simulink model "PMSM_PI"  (R2024a)
settings: Solver=FixedStepAuto  StartTime=0.0  StopTime=10  FixedStep=TsModel  RelTol=1e-3
values from neighbouring files (symbols this model uses):
  ADRC_times = 4.0    [data_PMSM_PI.sldd]
  B = 0.0    [data_PMSM_PI.sldd]
  b0 = 2000.0    [data_PMSM_PI.sldd]
  CCR_Counter = 4199.0    [data_PMSM_PI.sldd]
  CUR_I = 105.0    [data_PMSM_PI.sldd]
  CUR_P = 0.255    [data_PMSM_PI.sldd]
  current_bandwidth = 1500.0    [data_PMSM_PI.sldd]
  currunt_omega_c = 350.0    [data_PMSM_PI.sldd]
  flux = 0.00419    [data_PMSM_PI.sldd]
  Idq_limit = 20.0    [data_PMSM_PI.sldd]
  J = 5.8E-5    [data_PMSM_PI.sldd]
  Ld = 0.00017    [data_PMSM_PI.sldd]
  Lq = 0.00017    [data_PMSM_PI.sldd]
  Ls = 0.00017    [data_PMSM_PI.sldd]
  omega_c = 330.0    [data_PMSM_PI.sldd]
  omega_c_LQR = 35.0    [data_PMSM_PI.sldd]
  PMSM_CCR_Counter = 4199.0    [data_PMSM_PI.sldd]
  Pn = 5.0    [data_PMSM_PI.sldd]
  Rs = 0.07    [data_PMSM_PI.sldd]
  speed_bandwidth = 200.0    [data_PMSM_PI.sldd]
  speed_bandwidth_LQR = 60.0    [data_PMSM_PI.sldd]
  SPEED_I = 18.457    [data_PMSM_PI.sldd]
  SPEED_P = 0.18457    [data_PMSM_PI.sldd]
  Ts = 0.0001    [data_PMSM_PI.sldd]
  TsModel = 2.5E-5    [data_PMSM_PI.sldd]
  two_b0 = 2649534.0    [data_PMSM_PI.sldd]
  two_omega_c = 85.0    [data_PMSM_PI.sldd]
undefined symbols (not defined in the file or in its folder): DiscIntNeverNeededParam, sigbuilder_block
libraries: slpidlib x4, simulink x1, mcbplantlib x1, autolibpmsmexterior x1
(part 2 of 2)

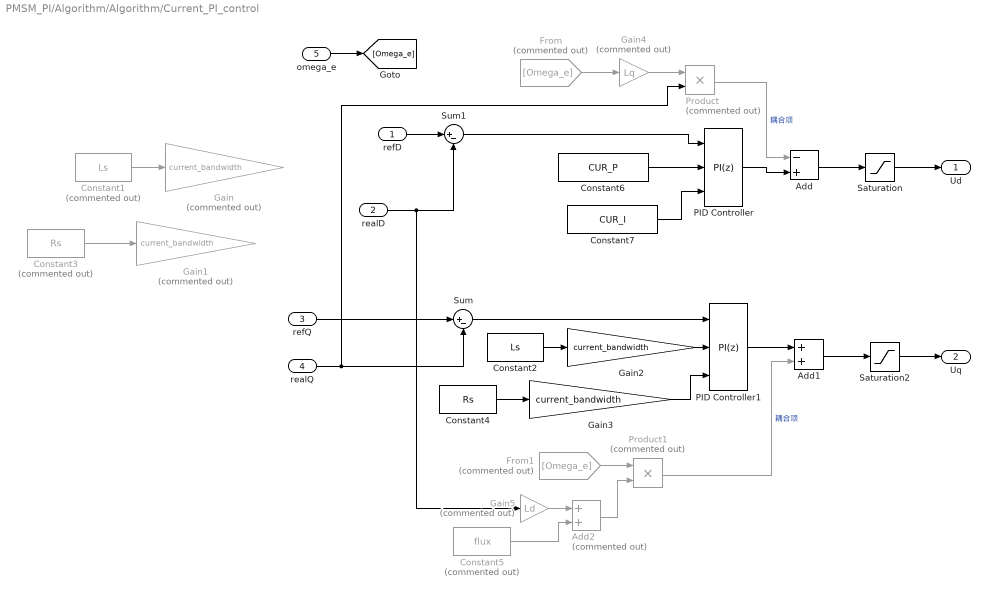
== system PMSM_PI/Algorithm/Algorithm/Current_PI_control ==
  refD : Inport  OutDataTypeStr=single
  realD : Inport  Port=2  OutDataTypeStr=single
  refQ : Inport  Port=3  OutDataTypeStr=single
  realQ : Inport  Port=4  OutDataTypeStr=single
  omega_e : Inport  Port=5  OutDataTypeStr=single
  Add : Sum  Inputs=-+  OutDataTypeStr=single
  Add1 : Sum  OutDataTypeStr=single
  Add2 : Sum  Commented=on  OutDataTypeStr=single
  Constant1 : Constant  Commented=on  Value=Ls  OutDataTypeStr=single  SampleTime=Ts
  Constant2 : Constant  Value=Ls  OutDataTypeStr=single  SampleTime=Ts
  Constant3 : Constant  Commented=on  Value=Rs  OutDataTypeStr=single  SampleTime=Ts
  Constant4 : Constant  Value=Rs  OutDataTypeStr=single  SampleTime=Ts
  Constant5 : Constant  Commented=on  Value=flux  OutDataTypeStr=single  SampleTime=Ts
  Constant6 : Constant  Value=CUR_P  OutDataTypeStr=single  SampleTime=Ts
  Constant7 : Constant  Value=CUR_I  OutDataTypeStr=single  SampleTime=Ts
  From : From  Commented=on  GotoTag=Omega_e
  From1 : From  Commented=on  GotoTag=Omega_e
  Gain : Gain  Commented=on  Gain=current_bandwidth  OutDataTypeStr=single
  Gain1 : Gain  Commented=on  Gain=current_bandwidth  OutDataTypeStr=single
  Gain2 : Gain  Gain=current_bandwidth  OutDataTypeStr=single
  Gain3 : Gain  Gain=current_bandwidth  OutDataTypeStr=single
  Gain4 : Gain  Commented=on  Gain=Lq  OutDataTypeStr=single
  Gain5 : Gain  Commented=on  Gain=Ld  OutDataTypeStr=single
  PID Controller : slpidlib/PID Controller  Controller=PI  Form=Parallel  TimeDomain=Discrete-time  UseExternalTs=off  SampleTime=Ts  IntegratorMethod=Forward Euler  FilterMethod=Forward Euler  ControllerParametersSource=external  P=1  I=1  UseKiTs=off  D=0  UseExternalDerivativeSource=off  N=100  UseFilter=on  TunerSelectOption=Transfer Function Based (PID Tuner App)  ZeroCross=off  InitialConditionSource=internal  InitialConditionForIntegrator=1  InitialConditionForFilter=0  DifferentiatorICPrevScaledInput=0  ExternalReset=none  TrackingMode=off  Kt=1  LimitOutput=off  SatLimitsSource=internal  UpperSaturationLimit=200  LowerSaturationLimit=-200  LinearizeAsGain=on  AntiWindupMode=none  Kb=1  LimitIntegrator=off  UpperIntegratorSaturationLimit=inf  LowerIntegratorSaturationLimit=-inf  POutMin=[]  POutMax=[]  IOutMin=[]  IOutMax=[]  DOutMin=[]  DOutMax=[]  NOutMin=[]  NOutMax=[]  SumOutMin=[]  SumOutMax=[]  SaturationOutMin=[]  SaturationOutMax=[]  PParamMin=[]  PParamMax=[]  IParamMin=[]  IParamMax=[]  DParamMin=[]  DParamMax=[]  NParamMin=[]  NParamMax=[]  KbParamMin=[]  KbParamMax=[]  KtParamMin=[]  KtParamMax=[]  KbOutMin=[]  KbOutMax=[]  KtOutMin=[]  KtOutMax=[]  IntegratorOutMin=[]  IntegratorOutMax=[]  FilterOutMin=[]  FilterOutMax=[]  SumI1OutMin=[]  SumI1OutMax=[]  SumI2OutMin=[]  SumI2OutMax=[]  SumI3OutMin=[]  SumI3OutMax=[]  SumI4OutMin=[]  SumI4OutMax=[]  SumDOutMin=[]  SumDOutMax=[]  DifferentiatorOutMin=[]  DifferentiatorOutMax=[]  FilterDiffOutCoefMin=[]  FilterDiffOutCoefMax=[]  ReciprocalOutMin=[]  ReciprocalOutMax=[]  SumDenOutMin=[]  SumDenOutMax=[]  SumNumOutMin=[]  SumNumOutMax=[]  DivideOutMin=[]  DivideOutMax=[]  UdiffTsProdOutMin=[]  UdiffTsProdOutMax=[]  NTsProdOutMin=[]  NTsProdOutMax=[]  UintegralTsProdOutMin=[]  UintegralTsProdOutMax=[]  UngainTsProdOutMin=[]  UngainTsProdOutMax=[]  ClampingZeroOutDataTypeStr=Inherit: Inherit via back propagation  ClampingZeroOutMin=[]  ClampingZeroOutMax=[]  FilterDenConstantOutDataTypeStr=Inherit: Inherit via back propagation  FilterDenConstantOutMin=[]  FilterDenConstantOutMax=[]  PCopyOutDataTypeStr=Inherit: Inherit via back propagation  PCopyOutMin=[]  PCopyOutMax=[]  NCopyOutDataTypeStr=Inherit: Inherit via back propagation  NCopyOutMin=[]  NCopyOutMax=[]  IntegratorContinuousStateAttributes=''  IntegratorStateMustResolveToSignalObject=off  IntegratorRTWStateStorageClass=Auto  FilterContinuousStateAttributes=''  FilterStateMustResolveToSignalObject=off  FilterRTWStateStorageClass=Auto  ParallelPVariant=ExternalParameters  IdealPVariant=Disabled  IVariant=ExternalParameters  DVariant=Disabled  IntegratorVariant=Discrete  SatVariant=Disabled  AWVariant=Passthrough  PCopyVariant=Disabled  TRVariant=Disabled  FdbkBlocksVariant=Forward  IdealPFdbkVariant=Disabled  SatFdbkVariant=Disabled  DerivativeFilterVariant=Disabled  NVariant=Disabled  NCopyVariant=Disabled_SignalSpec  FilterICVariant=Disabled  IntegratorICVariant=InternalICs  ExternalResetVariant=Disabled  TRSumVariant=Passthrough  SumFdbkVariant=Disabled  SumVariant=Sum_PI  TsampFilterVariant=InternalTs  TsampNgainVariant=Passthrough  TsampIntegralVariant=Disabled_SignalSpec  ExternalSaturationOutDataTypeStr=Inherit: Same as second input  DerivativeSourceVariant=Disabled
  PID Controller1 : slpidlib/PID Controller  Controller=PI  Form=Parallel  TimeDomain=Discrete-time  UseExternalTs=off  SampleTime=Ts  IntegratorMethod=Forward Euler  FilterMethod=Forward Euler  ControllerParametersSource=external  P=1  I=1  UseKiTs=off  D=0  UseExternalDerivativeSource=off  N=100  UseFilter=on  TunerSelectOption=Transfer Function Based (PID Tuner App)  ZeroCross=off  InitialConditionSource=internal  InitialConditionForIntegrator=1  InitialConditionForFilter=0  DifferentiatorICPrevScaledInput=0  ExternalReset=none  TrackingMode=off  Kt=1  LimitOutput=off  SatLimitsSource=internal  UpperSaturationLimit=200  LowerSaturationLimit=-200  LinearizeAsGain=on  AntiWindupMode=none  Kb=1  LimitIntegrator=off  UpperIntegratorSaturationLimit=inf  LowerIntegratorSaturationLimit=-inf  POutMin=[]  POutMax=[]  IOutMin=[]  IOutMax=[]  DOutMin=[]  DOutMax=[]  NOutMin=[]  NOutMax=[]  SumOutMin=[]  SumOutMax=[]  SaturationOutMin=[]  SaturationOutMax=[]  PParamMin=[]  PParamMax=[]  IParamMin=[]  IParamMax=[]  DParamMin=[]  DParamMax=[]  NParamMin=[]  NParamMax=[]  KbParamMin=[]  KbParamMax=[]  KtParamMin=[]  KtParamMax=[]  KbOutMin=[]  KbOutMax=[]  KtOutMin=[]  KtOutMax=[]  IntegratorOutMin=[]  IntegratorOutMax=[]  FilterOutMin=[]  FilterOutMax=[]  SumI1OutMin=[]  SumI1OutMax=[]  SumI2OutMin=[]  SumI2OutMax=[]  SumI3OutMin=[]  SumI3OutMax=[]  SumI4OutMin=[]  SumI4OutMax=[]  SumDOutMin=[]  SumDOutMax=[]  DifferentiatorOutMin=[]  DifferentiatorOutMax=[]  FilterDiffOutCoefMin=[]  FilterDiffOutCoefMax=[]  ReciprocalOutMin=[]  ReciprocalOutMax=[]  SumDenOutMin=[]  SumDenOutMax=[]  SumNumOutMin=[]  SumNumOutMax=[]  DivideOutMin=[]  DivideOutMax=[]  UdiffTsProdOutMin=[]  UdiffTsProdOutMax=[]  NTsProdOutMin=[]  NTsProdOutMax=[]  UintegralTsProdOutMin=[]  UintegralTsProdOutMax=[]  UngainTsProdOutMin=[]  UngainTsProdOutMax=[]  ClampingZeroOutDataTypeStr=Inherit: Inherit via back propagation  ClampingZeroOutMin=[]  ClampingZeroOutMax=[]  FilterDenConstantOutDataTypeStr=Inherit: Inherit via back propagation  FilterDenConstantOutMin=[]  FilterDenConstantOutMax=[]  PCopyOutDataTypeStr=Inherit: Inherit via back propagation  PCopyOutMin=[]  PCopyOutMax=[]  NCopyOutDataTypeStr=Inherit: Inherit via back propagation  NCopyOutMin=[]  NCopyOutMax=[]  IntegratorContinuousStateAttributes=''  IntegratorStateMustResolveToSignalObject=off  IntegratorRTWStateStorageClass=Auto  FilterContinuousStateAttributes=''  FilterStateMustResolveToSignalObject=off  FilterRTWStateStorageClass=Auto  ParallelPVariant=ExternalParameters  IdealPVariant=Disabled  IVariant=ExternalParameters  DVariant=Disabled  IntegratorVariant=Discrete  SatVariant=Disabled  AWVariant=Passthrough  PCopyVariant=Disabled  TRVariant=Disabled  FdbkBlocksVariant=Forward  IdealPFdbkVariant=Disabled  SatFdbkVariant=Disabled  DerivativeFilterVariant=Disabled  NVariant=Disabled  NCopyVariant=Disabled_SignalSpec  FilterICVariant=Disabled  IntegratorICVariant=InternalICs  ExternalResetVariant=Disabled  TRSumVariant=Passthrough  SumFdbkVariant=Disabled  SumVariant=Sum_PI  TsampFilterVariant=InternalTs  TsampNgainVariant=Passthrough  TsampIntegralVariant=Disabled_SignalSpec  ExternalSaturationOutDataTypeStr=Inherit: Same as second input  DerivativeSourceVariant=Disabled
  Product : Product  Commented=on  OutDataTypeStr=single
  Product1 : Product  Commented=on  OutDataTypeStr=single
  Saturation : Saturate  UpperLimit=Idq_limit  LowerLimit=-Idq_limit  OutDataTypeStr=single
  Saturation2 : Saturate  UpperLimit=Idq_limit  LowerLimit=-Idq_limit  OutDataTypeStr=single
  Sum : Sum  Inputs=|+-  OutDataTypeStr=single
  Sum1 : Sum  Inputs=|+-  OutDataTypeStr=single
  Ud : Outport  OutDataTypeStr=single
  Uq : Outport  Port=2  OutDataTypeStr=single
  wires:
  realD/1 -> Gain5/1, Sum1/2
  realQ/1 -> Product/2, Sum/2
  Add1/1 -> Saturation2/1
  Saturation/1 -> Ud/1
  Sum/1 -> PID Controller1/1
  Sum1/1 -> PID Controller/1
  refD/1 -> Sum1/1
  refQ/1 -> Sum/1
  Constant2/1 -> Gain2/1
  Gain3/1 -> PID Controller1/3
  Gain2/1 -> PID Controller1/2
  Constant1/1 -> Gain/1
  Constant4/1 -> Gain3/1
  Constant3/1 -> Gain1/1
  PID Controller/1 -> Add/2
  Add/1 -> Saturation/1
  omega_e/1 -> [Omega_e]
  From/1 -> Gain4/1
  Gain4/1 -> Product/1
  Product/1 -> Add/1  "耦合项"
  PID Controller1/1 -> Add1/1
  From1/1 -> Product1/1
  Gain5/1 -> Add2/1
  Constant5/1 -> Add2/2
  Add2/1 -> Product1/2
  Product1/1 -> Add1/2  "耦合项"
  Saturation2/1 -> Uq/1
  Constant6/1 -> PID Controller/2
  Constant7/1 -> PID Controller/3

== system PMSM_PI/Algorithm/Algorithm/Currunt_LADRC_Control ==
  Id_ref : Inport
  Id_real : Inport  Port=2
  Iq_ref : Inport  Port=3
  Iq_real : Inport  Port=4
  omega_e : Inport  Port=5
  Add3 : Sum  Inputs=-+  OutDataTypeStr=single
  Add4 : Sum  OutDataTypeStr=single
  Add5 : Sum  Commented=on  OutDataTypeStr=single
  Constant6 : Constant  Commented=on  Value=flux  OutDataTypeStr=single  SampleTime=Ts
  From12 : From  Commented=on  GotoTag=Omega_e
  From13 : From  Commented=on  GotoTag=Omega_e
  Gain6 : Gain  Commented=on  Gain=Lq  OutDataTypeStr=single
  Gain7 : Gain  Commented=on  Gain=Ld  OutDataTypeStr=single
  Id_Currunt_LADRC_Control : Subsystem
  Iq_Currunt_LADRC_Control : Subsystem
  Product2 : Product  Commented=on  OutDataTypeStr=single
  Product3 : Product  Commented=on  OutDataTypeStr=single
  Saturation1 : Saturate  UpperLimit=Idq_limit  LowerLimit=-Idq_limit  OutDataTypeStr=single
  Saturation3 : Saturate  UpperLimit=Idq_limit  LowerLimit=-Idq_limit  OutDataTypeStr=single
  ud_Ref : Outport
  uq_Ref : Outport  Port=2
  wires:
  Id_Currunt_LADRC_Control/1(ud_Ref) -> Add3/2
  Id_real/1 -> Gain7/1, Id_Currunt_LADRC_Control/2(Id_real)
  Product2/1 -> Add3/1  "耦合项"
  Constant6/1 -> Add5/2
  Product3/1 -> Add4/2  "耦合项"
  Id_ref/1 -> Id_Currunt_LADRC_Control/1(Id_ref)
  Add5/1 -> Product3/2
  Add3/1 -> Saturation1/1
  Iq_Currunt_LADRC_Control/1(uq_Ref) -> Add4/1
  Gain7/1 -> Add5/1
  Add4/1 -> Saturation3/1
  From12/1 -> Product3/1
  From13/1 -> Gain6/1
  Iq_ref/1 -> Iq_Currunt_LADRC_Control/1(Iq_ref)
  Iq_real/1 -> Product2/2, Iq_Currunt_LADRC_Control/2(Iq_real)
  Gain6/1 -> Product2/1
  Saturation1/1 -> ud_Ref/1
  Saturation3/1 -> uq_Ref/1
  omega_e/1 -> [Omega_e]

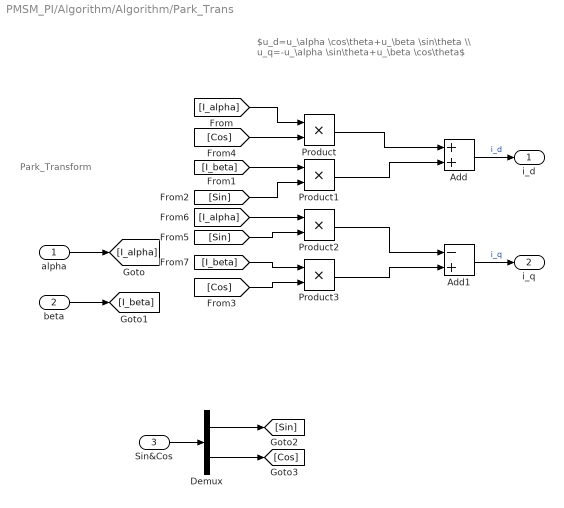
== system PMSM_PI/Algorithm/Algorithm/Park_Trans ==
  note: $u_d=u_\alpha \cos\theta+u_\beta \sin\theta \\ u_q=-u_\alpha \sin\theta+u_\beta \cos\theta$
  note: Park_Transform
  alpha : Inport  OutDataTypeStr=single
  beta : Inport  Port=2  OutDataTypeStr=single
  Sin&Cos : Inport  Port=3  OutDataTypeStr=single
  Add : Sum  OutDataTypeStr=single
  Add1 : Sum  Inputs=-+  OutDataTypeStr=single
  Demux : Demux  Outputs=2
  Product{,1..3} (4 alike) : Product  OutDataTypeStr=single
  i_d : Outport  OutDataTypeStr=single
  i_q : Outport  Port=2  OutDataTypeStr=single
  wires:
  Add1/1 -> i_q/1  "i_q"
  [Cos] -> Product/2
  Product/1 -> Add/1
  Product1/1 -> Add/2
  beta/1 -> [I_beta]
  Add/1 -> i_d/1  "i_d"
  [I_alpha] -> Product/1
  Product3/1 -> Add1/2
  [I_beta] -> Product3/1
  [I_beta] -> Product1/1
  [Sin] -> Product2/2
  Product2/1 -> Add1/1
  [Sin] -> Product1/2
  [I_alpha] -> Product2/1
  alpha/1 -> [I_alpha]
  [Cos] -> Product3/2
  Demux/1 -> [Sin]
  Demux/2 -> [Cos]
  Sin&Cos/1 -> Demux/1

== system PMSM_PI/Algorithm/Algorithm/SVPWM_By_Average_Zero_Injection ==
  d : Inport  OutDataTypeStr=single
  q : Inport  Port=2  OutDataTypeStr=single
  Sin&Cos : Inport  Port=3  OutDataTypeStr=single
  Udc : Inport  Port=4  OutDataTypeStr=single
  Anti_Park_Trans : Subsystem
  Gain : Gain  Gain=CCR_Counter  OutDataTypeStr=single
  Gain1 : Gain  Gain=CCR_Counter  OutDataTypeStr=single
  Gain2 : Gain  Gain=CCR_Counter  OutDataTypeStr=single
  SVPWM : Subsystem
  Scope : Scope  NumInputPorts=3
  Ta : Outport  OutDataTypeStr=single
  Tb : Outport  Port=2  OutDataTypeStr=single
  Tc : Outport  Port=3  OutDataTypeStr=single
  U_alpha : Outport  Port=4  OutDataTypeStr=single
  U_beta : Outport  Port=5  OutDataTypeStr=single
  wires:
  Anti_Park_Trans/1(alpha) -> U_alpha/1, SVPWM/1(alpha)
  q/1 -> Anti_Park_Trans/2(q)
  SVPWM/1(Ta) -> Scope/1, Gain/1
  Anti_Park_Trans/2(beta) -> U_beta/1, SVPWM/2(beta)
  d/1 -> Anti_Park_Trans/1(d)
  Sin&Cos/1 -> Anti_Park_Trans/3(Sin&Cos)
  SVPWM/2(Tb) -> Scope/2, Gain1/1
  SVPWM/3(Tc) -> Gain2/1, Scope/3
  Udc/1 -> SVPWM/3(Udc)
  Gain/1 -> Ta/1
  Gain1/1 -> Tb/1
  Gain2/1 -> Tc/1

== system PMSM_PI/Algorithm/Algorithm/Speed PI control2 ==
  Ref_RPM : Inport  OutDataTypeStr=single
  Real_RPM : Inport  Port=2  OutDataTypeStr=single
  Add : Sum  Inputs=+-  OutDataTypeStr=single
  Constant1 : Constant  Commented=on  Value=speed_bandwidth  OutDataTypeStr=single  SampleTime=Ts
  Constant2 : Constant  Value=speed_bandwidth  OutDataTypeStr=single  SampleTime=Ts
  Constant3 : Constant  Value=B  OutDataTypeStr=single  SampleTime=Ts
  Constant4 : Constant  Value=1.5*Pn*flux  OutDataTypeStr=single  SampleTime=Ts
  Constant5 : Constant  Value=SPEED_P  OutDataTypeStr=single  SampleTime=Ts
  Constant6 : Constant  Value=SPEED_I  OutDataTypeStr=single  SampleTime=Ts
  Divide : Product  Inputs=*/  OutDataTypeStr=single
  Gain : Gain  Commented=on  Gain=J/(1.5*Pn*flux)  OutDataTypeStr=single
  Gain1 : Gain  Commented=on  Gain=J/(1.5*Pn*flux)  OutDataTypeStr=single
  Gain2 : Gain  Gain=J  OutDataTypeStr=single
  PID Controller : slpidlib/PID Controller  Controller=PI  Form=Parallel  TimeDomain=Discrete-time  UseExternalTs=off  SampleTime=Ts  IntegratorMethod=Forward Euler  FilterMethod=Forward Euler  ControllerParametersSource=external  P=1  I=1  UseKiTs=off  D=0  UseExternalDerivativeSource=off  N=100  UseFilter=on  TunerSelectOption=Transfer Function Based (PID Tuner App)  ZeroCross=off  InitialConditionSource=internal  InitialConditionForIntegrator=1  InitialConditionForFilter=0  DifferentiatorICPrevScaledInput=0  ExternalReset=none  TrackingMode=off  Kt=1  LimitOutput=off  SatLimitsSource=internal  UpperSaturationLimit=200  LowerSaturationLimit=-200  LinearizeAsGain=on  AntiWindupMode=none  Kb=1  LimitIntegrator=off  UpperIntegratorSaturationLimit=inf  LowerIntegratorSaturationLimit=-inf  POutMin=[]  POutMax=[]  IOutMin=[]  IOutMax=[]  DOutMin=[]  DOutMax=[]  NOutMin=[]  NOutMax=[]  SumOutMin=[]  SumOutMax=[]  SaturationOutMin=[]  SaturationOutMax=[]  PParamMin=[]  PParamMax=[]  IParamMin=[]  IParamMax=[]  DParamMin=[]  DParamMax=[]  NParamMin=[]  NParamMax=[]  KbParamMin=[]  KbParamMax=[]  KtParamMin=[]  KtParamMax=[]  KbOutMin=[]  KbOutMax=[]  KtOutMin=[]  KtOutMax=[]  IntegratorOutMin=[]  IntegratorOutMax=[]  FilterOutMin=[]  FilterOutMax=[]  SumI1OutMin=[]  SumI1OutMax=[]  SumI2OutMin=[]  SumI2OutMax=[]  SumI3OutMin=[]  SumI3OutMax=[]  SumI4OutMin=[]  SumI4OutMax=[]  SumDOutMin=[]  SumDOutMax=[]  DifferentiatorOutMin=[]  DifferentiatorOutMax=[]  FilterDiffOutCoefMin=[]  FilterDiffOutCoefMax=[]  ReciprocalOutMin=[]  ReciprocalOutMax=[]  SumDenOutMin=[]  SumDenOutMax=[]  SumNumOutMin=[]  SumNumOutMax=[]  DivideOutMin=[]  DivideOutMax=[]  UdiffTsProdOutMin=[]  UdiffTsProdOutMax=[]  NTsProdOutMin=[]  NTsProdOutMax=[]  UintegralTsProdOutMin=[]  UintegralTsProdOutMax=[]  UngainTsProdOutMin=[]  UngainTsProdOutMax=[]  ClampingZeroOutDataTypeStr=Inherit: Inherit via back propagation  ClampingZeroOutMin=[]  ClampingZeroOutMax=[]  FilterDenConstantOutDataTypeStr=Inherit: Inherit via back propagation  FilterDenConstantOutMin=[]  FilterDenConstantOutMax=[]  PCopyOutDataTypeStr=Inherit: Inherit via back propagation  PCopyOutMin=[]  PCopyOutMax=[]  NCopyOutDataTypeStr=Inherit: Inherit via back propagation  NCopyOutMin=[]  NCopyOutMax=[]  IntegratorContinuousStateAttributes=''  IntegratorStateMustResolveToSignalObject=off  IntegratorRTWStateStorageClass=Auto  FilterContinuousStateAttributes=''  FilterStateMustResolveToSignalObject=off  FilterRTWStateStorageClass=Auto  ParallelPVariant=ExternalParameters  IdealPVariant=Disabled  IVariant=ExternalParameters  DVariant=Disabled  IntegratorVariant=Discrete  SatVariant=Disabled  AWVariant=Passthrough  PCopyVariant=Disabled  TRVariant=Disabled  FdbkBlocksVariant=Forward  IdealPFdbkVariant=Disabled  SatFdbkVariant=Disabled  DerivativeFilterVariant=Disabled  NVariant=Disabled  NCopyVariant=Disabled_SignalSpec  FilterICVariant=Disabled  IntegratorICVariant=InternalICs  ExternalResetVariant=Disabled  TRSumVariant=Passthrough  SumFdbkVariant=Disabled  SumVariant=Sum_PI  TsampFilterVariant=InternalTs  TsampNgainVariant=Passthrough  TsampIntegralVariant=Disabled_SignalSpec  ExternalSaturationOutDataTypeStr=Inherit: Same as second input  DerivativeSourceVariant=Disabled
  Product : Product  Commented=on  OutDataTypeStr=single
  Product1 : Product  OutDataTypeStr=single
  Saturation2 : Saturate  UpperLimit=Idq_limit  LowerLimit=-Idq_limit  OutDataTypeStr=single
  Sum1 : Sum  Inputs=|+-  OutDataTypeStr=single
  Sum2 : Sum  Inputs=|+-  OutDataTypeStr=single
  Iq_out : Outport  OutDataTypeStr=single
  wires:
  Constant1/1 -> Gain/1
  Ref_RPM/1 -> Sum1/1
  Sum1/1 -> PID Controller/1
  Real_RPM/1 -> Product1/2, Sum1/2
  PID Controller/1 -> Sum2/1
  Constant2/1 -> Product/1, Product/2, Gain2/1
  Product/1 -> Gain1/1
  Gain2/1 -> Add/1
  Constant3/1 -> Add/2
  Add/1 -> Divide/1
  Constant4/1 -> Divide/2
  Divide/1 -> Product1/1
  Product1/1 -> Sum2/2
  Saturation2/1 -> Iq_out/1
  Sum2/1 -> Saturation2/1
  Constant5/1 -> PID Controller/2
  Constant6/1 -> PID Controller/3

== system PMSM_PI/Algorithm/Algorithm/Speed SMC control1 ==
  note: 机械转速（rad/s）
  note: 转速值（单位RPM）
  Ref_RPM : Inport  OutDataTypeStr=single
  Real_RPM : Inport  Port=2  OutDataTypeStr=single
  1/D : Gain  Gain=1/(1.5*Pn*flux/2/J)  SaturateOnIntegerOverflow=on  SampleTime=Ts  OutDataTypeStr=Inherit: Same as input  ParamDataTypeStr=Inherit: Same as input
  Discrete Derivative : simulink/Discrete/Discrete Derivative  gainval=1.0  ICPrevScaledInput=0.0  OutMin=[]  OutMax=[]  OutDataType=fixdt(1, 16)  OutScaling=2^-10  DoSatur=off
  Discrete-Time Integrator : DiscreteIntegrator  InitialCondition=0.001  SampleTime=Ts  ICPrevOutput=DiscIntNeverNeededParam  ICPrevScaledInput=DiscIntNeverNeededParam
  Kp1 : Gain  Gain=300  SaturateOnIntegerOverflow=on  SampleTime=Ts  OutDataTypeStr=Inherit: Same as input  ParamDataTypeStr=Inherit: Same as input
  Kp2 : Gain  Gain=200  SaturateOnIntegerOverflow=on  SampleTime=Ts  OutDataTypeStr=Inherit: Same as input  ParamDataTypeStr=Inherit: Same as input
  Kp3 : Gain  Gain=60  SaturateOnIntegerOverflow=on  SampleTime=Ts  OutDataTypeStr=Inherit: Same as input  ParamDataTypeStr=Inherit: Same as input
  Kp4 : Gain  Gain=60  SaturateOnIntegerOverflow=on  SampleTime=Ts  OutDataTypeStr=Inherit: Same as input  ParamDataTypeStr=Inherit: Same as input
  Nr->wm : Gain  Gain=pi/30  SaturateOnIntegerOverflow=on  SampleTime=Ts  OutDataTypeStr=Inherit: Same as input  ParamDataTypeStr=Inherit: Same as input
  Saturation2 : Saturate  UpperLimit=Idq_limit  LowerLimit=-Idq_limit  OutDataTypeStr=single
  Sign : Signum
  Sum1 : Sum  Inputs=|+-  OutDataTypeStr=single
  Sum3 : Sum  InputSameDT=on  SaturateOnIntegerOverflow=on  SampleTime=Ts  OutDataTypeStr=Inherit: Same as first input
  Sum4 : Sum  Inputs=++-  InputSameDT=on  SaturateOnIntegerOverflow=on  SampleTime=Ts  OutDataTypeStr=Inherit: Same as first input
  Iq_out : Outport  OutDataTypeStr=single
  wires:
  Ref_RPM/1 -> Sum1/1
  Real_RPM/1 -> Sum1/2
  Saturation2/1 -> Iq_out/1
  Discrete-Time Integrator/1 -> 1/D/1
  Sign/1 -> Kp2/1
  Kp1/1 -> Sum4/1
  Kp3/1 -> Sum4/3
  Kp4/1 -> Sum3/1
  Sum4/1 -> Discrete-Time Integrator/1
  Sum1/1 -> Nr->wm/1
  Sum3/1 -> Sign/1, Kp1/1
  Discrete Derivative/1 -> Kp3/1, Sum3/2  "x2"
  Kp2/1 -> Sum4/2
  Nr->wm/1 -> Discrete Derivative/1, Kp4/1  "x1"
  1/D/1 -> Saturation2/1

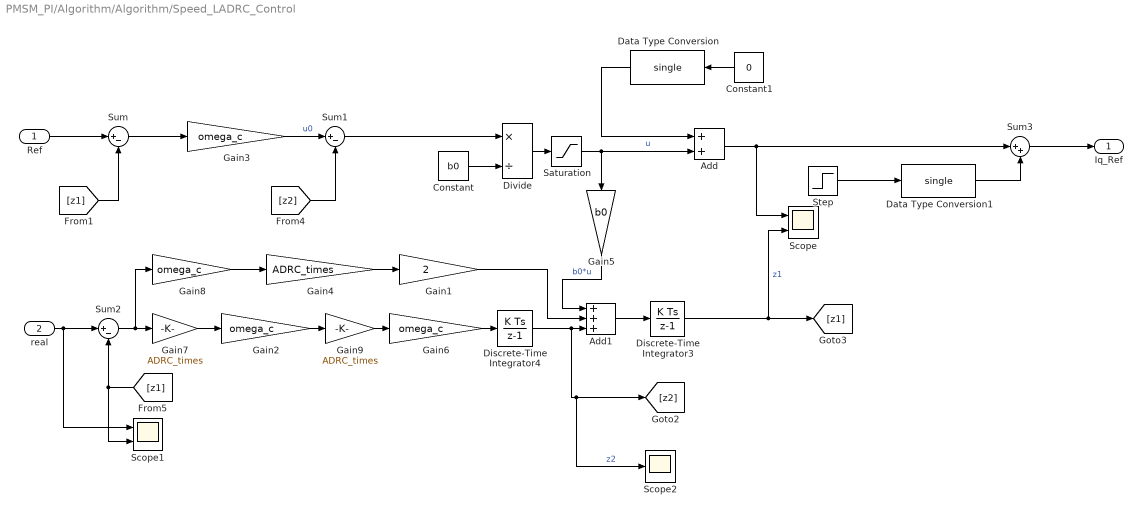
== system PMSM_PI/Algorithm/Algorithm/Speed_LADRC_Control ==
  Ref : Inport  OutDataTypeStr=single
  real : Inport  Port=2  OutDataTypeStr=single
  Add : Sum  OutDataTypeStr=single
  Add1 : Sum  Inputs=+++  OutDataTypeStr=single
  Constant : Constant  Value=b0  OutDataTypeStr=single
  Constant1 : Constant  Value=0  SampleTime=-1
  Data Type Conversion : DataTypeConversion  OutDataTypeStr=single  SaturateOnIntegerOverflow=off  RndMeth=Floor
  Data Type Conversion1 : DataTypeConversion  OutDataTypeStr=single  SaturateOnIntegerOverflow=off  RndMeth=Floor
  Discrete-Time Integrator3 : DiscreteIntegrator  SampleTime=-1  OutDataTypeStr=single  ICPrevOutput=DiscIntNeverNeededParam  ICPrevScaledInput=DiscIntNeverNeededParam
  Discrete-Time Integrator4 : DiscreteIntegrator  SampleTime=-1  OutDataTypeStr=single  ICPrevOutput=DiscIntNeverNeededParam  ICPrevScaledInput=DiscIntNeverNeededParam
  Divide : Product  Inputs=*/  OutDataTypeStr=single
  Gain1 : Gain  Gain=2  OutDataTypeStr=single
  Gain{2..3,6,8} (4 alike) : Gain  Gain=omega_c  OutDataTypeStr=single
  Gain4 : Gain  Gain=ADRC_times  OutDataTypeStr=single
  Gain5 : Gain  Gain=b0  OutDataTypeStr=single
  Gain7 : Gain  Gain=ADRC_times  OutDataTypeStr=single
  Gain9 : Gain  Gain=ADRC_times  OutDataTypeStr=single
  Saturation : Saturate  UpperLimit=Idq_limit  LowerLimit=-Idq_limit  OutDataTypeStr=single
  Scope : Scope  NumInputPorts=2
  Scope1 : Scope  NumInputPorts=2
  Scope2 : Scope
  Step : Step  Time=8  SampleTime=0
  Sum : Sum  Inputs=|+-  OutDataTypeStr=single
  Sum1 : Sum  Inputs=|+-  OutDataTypeStr=single
  Sum2 : Sum  Inputs=|+-  OutDataTypeStr=single
  Sum3 : Sum  Inputs=|++
  Iq_Ref : Outport  OutDataTypeStr=single
  wires:
  Ref/1 -> Sum/1
  Discrete-Time Integrator4/1 -> Add1/3, Scope2/1, [z2]  "z2"
  Gain5/1 -> Add1/1  "b0*u"
  Gain2/1 -> Gain9/1
  Gain1/1 -> Add1/2
  Discrete-Time Integrator3/1 -> Scope/2, [z1]  "z1"
  Add1/1 -> Discrete-Time Integrator3/1
  Sum2/1 -> Gain7/1, Gain8/1
  real/1 -> Scope1/1, Sum2/1
  [z1] -> Scope1/2, Sum2/2
  [z1] -> Sum/2
  Sum/1 -> Gain3/1
  [z2] -> Sum1/2
  Constant/1 -> Divide/2
  Divide/1 -> Saturation/1
  Gain3/1 -> Sum1/1  "u0"
  Sum1/1 -> Divide/1
  Add/1 -> Scope/1, Sum3/1
  Data Type Conversion/1 -> Add/1
  Saturation/1 -> Add/2, Gain5/1  "u"
  Gain4/1 -> Gain1/1
  Gain6/1 -> Discrete-Time Integrator4/1
  Gain7/1 -> Gain2/1
  Gain8/1 -> Gain4/1
  Gain9/1 -> Gain6/1
  Constant1/1 -> Data Type Conversion/1
  Sum3/1 -> Iq_Ref/1
  Step/1 -> Data Type Conversion1/1
  Data Type Conversion1/1 -> Sum3/2

== system PMSM_PI/Algorithm/Algorithm/Subsystem1 ==
  rpm_ref : Inport
  rpm_real : Inport  Port=2
  Id_ref : Inport  Port=3
  Id_real : Inport  Port=4
  Id_Currunt_LADRC_Control : Subsystem
  Subsystem : Subsystem
  uq_ref : Outport
  ud_Ref : Outport  Port=2
  wires:
  Id_Currunt_LADRC_Control/1(ud_Ref) -> ud_Ref/1
  Id_real/1 -> Id_Currunt_LADRC_Control/2(Id_real)
  Id_ref/1 -> Id_Currunt_LADRC_Control/1(Id_ref)
  rpm_ref/1 -> Subsystem/1(rpm_ref)
  rpm_real/1 -> Subsystem/2(rpm_real)
  Subsystem/1(uq_ref) -> uq_ref/1

== system PMSM_PI/Algorithm/Algorithm/Theta_to_SinCos ==
  Theta_in : Inport  OutDataTypeStr=single
  Mux : Mux  Inputs=2
  Sin : Trigonometry
  Sin1 : Trigonometry  Operator=cos
  Sin&Cos : Outport  OutDataTypeStr=single
  wires:
  Theta_in/1 -> Sin1/1, Sin/1
  Sin/1 -> Mux/1
  Sin1/1 -> Mux/2
  Mux/1 -> Sin&Cos/1

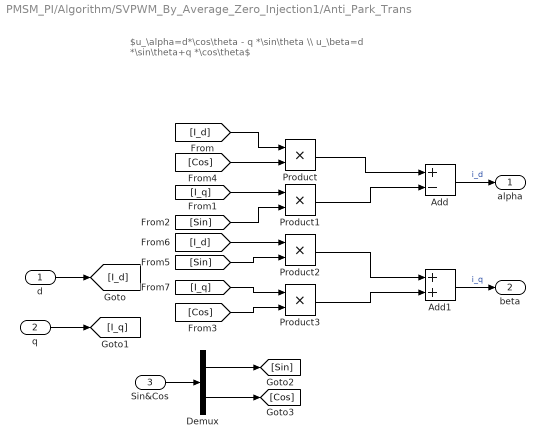
== system PMSM_PI/Algorithm/SVPWM_By_Average_Zero_Injection1/Anti_Park_Trans ==
  note: $u_\alpha=d*\cos\theta - q *\sin\theta \\ u_\beta=d *\sin\theta+q *\cos\theta$
  d : Inport  OutDataTypeStr=single
  q : Inport  Port=2  OutDataTypeStr=single
  Sin&Cos : Inport  Port=3  OutDataTypeStr=single
  Add : Sum  Inputs=+-  OutDataTypeStr=single
  Add1 : Sum  OutDataTypeStr=single
  Demux : Demux  Outputs=2
  Product{,1..3} (4 alike) : Product  OutDataTypeStr=single
  alpha : Outport  OutDataTypeStr=single
  beta : Outport  Port=2  OutDataTypeStr=single
  wires:
  Add1/1 -> beta/1  "i_q"
  Sin&Cos/1 -> Demux/1
  [Cos] -> Product/2
  Product/1 -> Add/1
  Product1/1 -> Add/2
  q/1 -> [I_q]
  Add/1 -> alpha/1  "i_d"
  [I_d] -> Product/1
  Product3/1 -> Add1/2
  [I_q] -> Product3/1
  [I_q] -> Product1/1
  [Sin] -> Product2/2
  Product2/1 -> Add1/1
  [Sin] -> Product1/2
  [I_d] -> Product2/1
  d/1 -> [I_d]
  [Cos] -> Product3/2
  Demux/1 -> [Sin]
  Demux/2 -> [Cos]

== system PMSM_PI/Algorithm/SVPWM_By_Average_Zero_Injection1/SVPWM ==
  alpha : Inport  OutDataTypeStr=single
  beta : Inport  Port=2  OutDataTypeStr=single
  Udc : Inport  Port=3  OutDataTypeStr=single
  Add{,1..4} (5 alike) : Sum  OutDataTypeStr=single
  Anti_Clark_Trans : Subsystem
  Constant : Constant  Value=0.5  OutDataTypeStr=single  SampleTime=Ts
  Demux : Demux  Outputs=3
  Divide : Product  Inputs=*/  OutDataTypeStr=single
  Gain : Gain  Gain=-0.5  OutDataTypeStr=single
  Gain1 : Gain  Gain=-1
  Max : MinMax  Function=max  Inputs=3  OutDataTypeStr=single
  Max1 : MinMax  Inputs=3  OutDataTypeStr=single
  Mux : Mux  Inputs=3
  Scope : Scope  NumInputPorts=3
  Ta : Outport  OutDataTypeStr=single
  Tb : Outport  Port=2  OutDataTypeStr=single
  Tc : Outport  Port=3  OutDataTypeStr=single
  wires:
  Anti_Clark_Trans/1(A) -> Max1/1, Max/1, Add/1
  Gain/1 -> Add/2, Add1/2, Add2/2
  Anti_Clark_Trans/2(B) -> Max1/2, Max/2, Add1/1
  Anti_Clark_Trans/3(C) -> Max1/3, Max/3, Add2/1
  Add3/1 -> Gain/1
  Max/1 -> Add3/1
  alpha/1 -> Anti_Clark_Trans/1(alpha)
  beta/1 -> Anti_Clark_Trans/2(beta)
  Add/1 -> Mux/1
  Add1/1 -> Mux/2
  Add2/1 -> Mux/3
  Mux/1 -> Gain1/1
  Demux/1 -> Ta/1
  Demux/2 -> Tb/1
  Demux/3 -> Tc/1
  Divide/1 -> Scope/2, Add4/1
  Constant/1 -> Add4/2
  Max1/1 -> Add3/2
  Udc/1 -> Divide/2
  Add4/1 -> Demux/1, Scope/3
  Gain1/1 -> Scope/1, Divide/1

== system PMSM_PI/Algorithm/Algorithm/Currunt_LADRC_Control/Id_Currunt_LADRC_Control ==
  Id_ref : Inport
  Id_real : Inport  Port=2
  Add1 : Sum  Inputs=+++
  Constant : Constant  Value=b0
  Data Type Conversion : DataTypeConversion  OutDataTypeStr=single  SaturateOnIntegerOverflow=off  RndMeth=Floor
  Discrete-Time Integrator3 : DiscreteIntegrator  SampleTime=-1  ICPrevOutput=DiscIntNeverNeededParam  ICPrevScaledInput=DiscIntNeverNeededParam
  Discrete-Time Integrator4 : DiscreteIntegrator  SampleTime=-1  ICPrevOutput=DiscIntNeverNeededParam  ICPrevScaledInput=DiscIntNeverNeededParam
  Divide : Product  Inputs=*/
  Gain1 : Gain  Gain=2*ADRC_times*omega_c
  Gain2 : Gain  Gain=ADRC_times*ADRC_times*omega_c*omega_c
  Gain3 : Gain  Gain=omega_c
  Gain5 : Gain  Gain=b0
  Scope2 : Scope
  Sum : Sum  Inputs=|+-
  Sum1 : Sum  Inputs=|+-
  Sum2 : Sum  Inputs=|+-
  ud_Ref : Outport
  wires:
  Sum1/1 -> Divide/1
  Gain3/1 -> Sum1/1  "u"
  Divide/1 -> Gain5/1, ud_Ref/1
  Constant/1 -> Data Type Conversion/1
  [z2] -> Sum1/2
  Sum/1 -> Gain3/1
  [z1] -> Sum/2
  [z1] -> Sum2/2
  Id_real/1 -> Sum2/1
  Add1/1 -> Discrete-Time Integrator3/1
  Discrete-Time Integrator3/1 -> [z1]  "z1"
  Gain1/1 -> Add1/2
  Gain2/1 -> Discrete-Time Integrator4/1
  Gain5/1 -> Add1/1  "u"
  Discrete-Time Integrator4/1 -> Scope2/1, [z2], Add1/3  "z2"
  Id_ref/1 -> Sum/1
  Data Type Conversion/1 -> Divide/2
  Sum2/1 -> Gain1/1, Gain2/1

== system PMSM_PI/Algorithm/Algorithm/Currunt_LADRC_Control/Iq_Currunt_LADRC_Control ==
  Iq_ref : Inport
  Iq_real : Inport  Port=2
  Add1 : Sum  Inputs=+++
  Constant : Constant  Value=b0
  Data Type Conversion : DataTypeConversion  OutDataTypeStr=single  SaturateOnIntegerOverflow=off  RndMeth=Floor
  Discrete-Time Integrator3 : DiscreteIntegrator  SampleTime=-1  ICPrevOutput=DiscIntNeverNeededParam  ICPrevScaledInput=DiscIntNeverNeededParam
  Discrete-Time Integrator4 : DiscreteIntegrator  SampleTime=-1  ICPrevOutput=DiscIntNeverNeededParam  ICPrevScaledInput=DiscIntNeverNeededParam
  Divide : Product  Inputs=*/
  Gain1 : Gain  Gain=2*ADRC_times*omega_c
  Gain2 : Gain  Gain=ADRC_times*ADRC_times*omega_c*omega_c
  Gain3 : Gain  Gain=omega_c
  Gain5 : Gain  Gain=b0
  Scope2 : Scope
  Sum : Sum  Inputs=|+-
  Sum1 : Sum  Inputs=|+-
  Sum2 : Sum  Inputs=|+-
  uq_Ref : Outport
  wires:
  Iq_ref/1 -> Sum/1
  Discrete-Time Integrator4/1 -> Add1/3, [z2], Scope2/1  "z2"
  Gain5/1 -> Add1/1  "u"
  Gain2/1 -> Discrete-Time Integrator4/1
  Gain1/1 -> Add1/2
  Discrete-Time Integrator3/1 -> [z1]  "z1"
  Add1/1 -> Discrete-Time Integrator3/1
  Sum2/1 -> Gain2/1, Gain1/1
  Iq_real/1 -> Sum2/1
  [z1] -> Sum2/2
  [z1] -> Sum/2
  Sum/1 -> Gain3/1
  [z2] -> Sum1/2
  Constant/1 -> Data Type Conversion/1
  Divide/1 -> uq_Ref/1, Gain5/1
  Gain3/1 -> Sum1/1  "u"
  Sum1/1 -> Divide/1
  Data Type Conversion/1 -> Divide/2

== system PMSM_PI/Algorithm/Algorithm/SVPWM_By_Average_Zero_Injection/Anti_Park_Trans ==
  note: $u_\alpha=d*\cos\theta - q *\sin\theta \\ u_\beta=d *\sin\theta+q *\cos\theta$
  d : Inport  OutDataTypeStr=single
  q : Inport  Port=2  OutDataTypeStr=single
  Sin&Cos : Inport  Port=3  OutDataTypeStr=single
  Add : Sum  Inputs=+-  OutDataTypeStr=single
  Add1 : Sum  OutDataTypeStr=single
  Demux : Demux  Outputs=2
  Product{,1..3} (4 alike) : Product  OutDataTypeStr=single
  alpha : Outport  OutDataTypeStr=single
  beta : Outport  Port=2  OutDataTypeStr=single
  wires:
  Add1/1 -> beta/1  "i_q"
  Sin&Cos/1 -> Demux/1
  [Cos] -> Product/2
  Product/1 -> Add/1
  Product1/1 -> Add/2
  q/1 -> [I_q]
  Add/1 -> alpha/1  "i_d"
  [I_d] -> Product/1
  Product3/1 -> Add1/2
  [I_q] -> Product3/1
  [I_q] -> Product1/1
  [Sin] -> Product2/2
  Product2/1 -> Add1/1
  [Sin] -> Product1/2
  [I_d] -> Product2/1
  d/1 -> [I_d]
  [Cos] -> Product3/2
  Demux/1 -> [Sin]
  Demux/2 -> [Cos]

== system PMSM_PI/Algorithm/Algorithm/SVPWM_By_Average_Zero_Injection/SVPWM ==
  alpha : Inport  OutDataTypeStr=single
  beta : Inport  Port=2  OutDataTypeStr=single
  Udc : Inport  Port=3  OutDataTypeStr=single
  Add{,1..4} (5 alike) : Sum  OutDataTypeStr=single
  Anti_Clark_Trans : Subsystem
  Constant : Constant  Value=0.5  OutDataTypeStr=single  SampleTime=Ts
  Demux : Demux  Outputs=3
  Divide : Product  Inputs=*/  OutDataTypeStr=single
  Gain : Gain  Gain=-0.5  OutDataTypeStr=single
  Gain1 : Gain  Gain=-1
  Max : MinMax  Function=max  Inputs=3  OutDataTypeStr=single
  Max1 : MinMax  Inputs=3  OutDataTypeStr=single
  Mux : Mux  Inputs=3
  Scope : Scope  NumInputPorts=3
  Ta : Outport  OutDataTypeStr=single
  Tb : Outport  Port=2  OutDataTypeStr=single
  Tc : Outport  Port=3  OutDataTypeStr=single
  wires:
  Anti_Clark_Trans/1(A) -> Max1/1, Max/1, Add/1
  Gain/1 -> Add/2, Add1/2, Add2/2
  Anti_Clark_Trans/2(B) -> Max1/2, Max/2, Add1/1
  Anti_Clark_Trans/3(C) -> Max1/3, Max/3, Add2/1
  Add3/1 -> Gain/1
  Max/1 -> Add3/1
  alpha/1 -> Anti_Clark_Trans/1(alpha)
  beta/1 -> Anti_Clark_Trans/2(beta)
  Add/1 -> Mux/1
  Add1/1 -> Mux/2
  Add2/1 -> Mux/3
  Mux/1 -> Gain1/1
  Demux/1 -> Ta/1
  Demux/2 -> Tb/1
  Demux/3 -> Tc/1
  Divide/1 -> Scope/2, Add4/1
  Constant/1 -> Add4/2
  Max1/1 -> Add3/2
  Udc/1 -> Divide/2
  Add4/1 -> Demux/1, Scope/3
  Gain1/1 -> Scope/1, Divide/1

== system PMSM_PI/Algorithm/Algorithm/Subsystem1/Id_Currunt_LADRC_Control ==
  Id_ref : Inport
  Id_real : Inport  Port=2
  Add1 : Sum  Inputs=+++
  Constant : Constant  Value=b0
  Data Type Conversion : DataTypeConversion  OutDataTypeStr=single  SaturateOnIntegerOverflow=off  RndMeth=Floor
  Discrete-Time Integrator3 : DiscreteIntegrator  SampleTime=-1  ICPrevOutput=DiscIntNeverNeededParam  ICPrevScaledInput=DiscIntNeverNeededParam
  Discrete-Time Integrator4 : DiscreteIntegrator  SampleTime=-1  ICPrevOutput=DiscIntNeverNeededParam  ICPrevScaledInput=DiscIntNeverNeededParam
  Divide : Product  Inputs=*/
  Gain : Gain  Gain=currunt_omega_c
  Gain1 : Gain  Gain=2*ADRC_times*currunt_omega_c
  Gain2 : Gain  Gain=ADRC_times*ADRC_times*currunt_omega_c*currunt_omega_c
  Gain5 : Gain  Gain=b0
  Saturation2 : Saturate  UpperLimit=Idq_limit  LowerLimit=-Idq_limit  OutDataTypeStr=single
  Scope2 : Scope
  Sum : Sum  Inputs=|+-
  Sum1 : Sum  Inputs=|+-
  Sum2 : Sum  Inputs=|+-
  ud_Ref : Outport
  wires:
  Sum1/1 -> Divide/1
  Gain/1 -> Sum1/1  "u"
  Divide/1 -> Gain5/1, Saturation2/1
  Constant/1 -> Data Type Conversion/1
  [z2] -> Sum1/2
  Sum/1 -> Gain/1
  [z1] -> Sum/2
  [z1] -> Sum2/2
  Id_real/1 -> Sum2/1
  Add1/1 -> Discrete-Time Integrator3/1
  Discrete-Time Integrator3/1 -> [z1]  "z1"
  Gain1/1 -> Add1/2
  Gain2/1 -> Discrete-Time Integrator4/1
  Gain5/1 -> Add1/1  "u"
  Discrete-Time Integrator4/1 -> Scope2/1, [z2], Add1/3  "z2"
  Id_ref/1 -> Sum/1
  Data Type Conversion/1 -> Divide/2
  Sum2/1 -> Gain1/1, Gain2/1
  Saturation2/1 -> ud_Ref/1

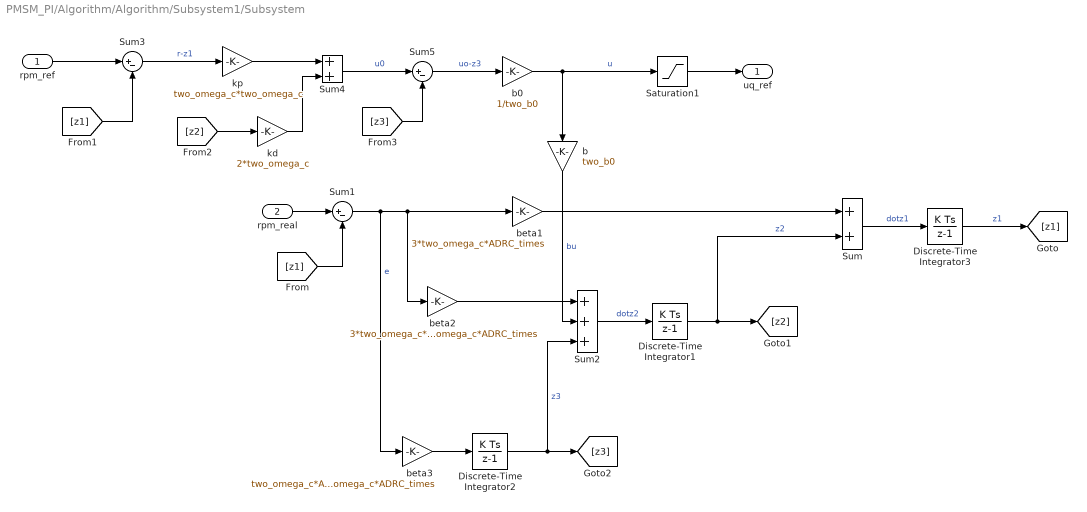
== system PMSM_PI/Algorithm/Algorithm/Subsystem1/Subsystem ==
  rpm_ref : Inport
  rpm_real : Inport  Port=2
  Discrete-Time Integrator1 : DiscreteIntegrator  SampleTime=-1  ICPrevOutput=DiscIntNeverNeededParam  ICPrevScaledInput=DiscIntNeverNeededParam
  Discrete-Time Integrator2 : DiscreteIntegrator  SampleTime=-1  ICPrevOutput=DiscIntNeverNeededParam  ICPrevScaledInput=DiscIntNeverNeededParam
  Discrete-Time Integrator3 : DiscreteIntegrator  SampleTime=-1  ICPrevOutput=DiscIntNeverNeededParam  ICPrevScaledInput=DiscIntNeverNeededParam
  Saturation1 : Saturate  UpperLimit=Idq_limit  LowerLimit=-Idq_limit  OutDataTypeStr=single
  Sum : Sum
  Sum1 : Sum  Inputs=|+-
  Sum2 : Sum  Inputs=+++
  Sum3 : Sum  Inputs=|+-
  Sum4 : Sum
  Sum5 : Sum  Inputs=|+-
  b : Gain  Gain=two_b0
  b0 : Gain  Gain=1/two_b0
  beta1 : Gain  Gain=3*two_omega_c*ADRC_times
  beta2 : Gain  Gain=3*two_omega_c*ADRC_times*two_omega_c*ADRC_times
  beta3 : Gain  Gain=two_omega_c*ADRC_times*two_omega_c*ADRC_times*two_omega_c*ADRC_times
  kd : Gain  Gain=2*two_omega_c
  kp : Gain  Gain=two_omega_c*two_omega_c
  uq_ref : Outport
  wires:
  Sum1/1 -> beta1/1, beta2/1, beta3/1  "e"
  Sum2/1 -> Discrete-Time Integrator1/1  "dotz2"
  beta3/1 -> Discrete-Time Integrator2/1
  [z3] -> Sum5/2
  b/1 -> Sum2/2  "bu"
  Discrete-Time Integrator3/1 -> [z1]  "z1"
  Sum5/1 -> b0/1  "uo-z3"
  Discrete-Time Integrator1/1 -> Sum/2, [z2]  "z2"
  [z1] -> Sum1/2
  Discrete-Time Integrator2/1 -> Sum2/3, [z3]  "z3"
  Sum4/1 -> Sum5/1  "u0"
  Sum3/1 -> kp/1  "r-z1"
  [z1] -> Sum3/2
  rpm_ref/1 -> Sum3/1
  beta2/1 -> Sum2/1
  [z2] -> kd/1
  rpm_real/1 -> Sum1/1
  b0/1 -> b/1, Saturation1/1  "u"
  kp/1 -> Sum4/1
  kd/1 -> Sum4/2
  Sum/1 -> Discrete-Time Integrator3/1  "dotz1"
  Saturation1/1 -> uq_ref/1
  beta1/1 -> Sum/1

== system PMSM_PI/Algorithm/SVPWM_By_Average_Zero_Injection1/SVPWM/Anti_Clark_Trans ==
  alpha : Inport  OutDataTypeStr=single
  beta : Inport  Port=2  OutDataTypeStr=single
  Add : Sum  Inputs=-+  OutDataTypeStr=single
  Add1 : Sum  Inputs=--  OutDataTypeStr=single
  Gain : Gain  Gain=0.5  OutDataTypeStr=single
  Gain1 : Gain  Gain=sqrt(3)/2  OutDataTypeStr=single
  A : Outport  OutDataTypeStr=single
  B : Outport  Port=2  OutDataTypeStr=single
  C : Outport  Port=3  OutDataTypeStr=single
  wires:
  Add1/1 -> C/1
  Gain/1 -> Add1/1, Add/1
  Add/1 -> B/1
  alpha/1 -> A/1, Gain/1
  Gain1/1 -> Add1/2, Add/2
  beta/1 -> Gain1/1

== system PMSM_PI/Algorithm/Algorithm/SVPWM_By_Average_Zero_Injection/SVPWM/Anti_Clark_Trans ==
  alpha : Inport  OutDataTypeStr=single
  beta : Inport  Port=2  OutDataTypeStr=single
  Add : Sum  Inputs=-+  OutDataTypeStr=single
  Add1 : Sum  Inputs=--  OutDataTypeStr=single
  Gain : Gain  Gain=0.5  OutDataTypeStr=single
  Gain1 : Gain  Gain=sqrt(3)/2  OutDataTypeStr=single
  A : Outport  OutDataTypeStr=single
  B : Outport  Port=2  OutDataTypeStr=single
  C : Outport  Port=3  OutDataTypeStr=single
  wires:
  Add1/1 -> C/1
  Gain/1 -> Add1/1, Add/1
  Add/1 -> B/1
  alpha/1 -> A/1, Gain/1
  Gain1/1 -> Add1/2, Add/2
  beta/1 -> Gain1/1

== matlab function PMSM_PI/Algorithm/双环LQR/MATLAB Function2 ==
  data: P input; k output; Flux input; J input; Rs input; Ls input; B input; we input
function k  = fcn(P,Flux,J,Rs,Ls,B,we)

%A = [1-T*B/J 0 T*3*P*Flux/2/J;0 1-T-Rs/Ls T*we;-T*P*Flux/Ls -T*we 1-T*Rs/Ls];  %3*3
%B = [0 0;T/Ls 0;0 T/Ls];  %3*2
A = [-B/J 0 3*P*Flux/2/J;0 -Rs/Ls we;-P*Flux/Ls -we -Rs/Ls];  %3*3
B = [0 0;1/Ls 0;0 1/Ls];  %3*2
C = [1 0 0;0 1 0;0 0 1];  %3*3
D = 0;  %3*2  zeros(3,2)

Q = [100 0 0;0 10 0;0 0 10];  %3*3
R = [0.1 0;0 0.1];  %2*2

%X0=[];
N = 5;  %迭代次数
P = zeros(3,3,N+1);  %P的初始化,N+1个3*3的二维数组
P(:,:,N+1) = Q; %P的最后一个值为Q  P(:,:,2)=Q

for t=2:(N+1)  %t从2到21
    tused = (N+3-t);  %tused从21到2
    P(:,:,tused-1) = Q + A'*P(:,:,tused)*A-A'*P(:,:,tused)*B/(R+B'*P(:,:,tused)*B)*B'*P(:,:,tused)*A;  %黎卡提方程P的值为3*3   P(:,:,1)
end

K = zeros(2,3,N);  %初始化20*3

%U = zeros(N,2);  %初始化20*2
%X(1,:) = X0;

for t=1:N  %从1到20
K(:,:,t)=-(R+B'*P(:,:,t+1)*B)\B'*P(:,:,t+1)*A; %2*3
%U(t,:)=K(t,:)*X(t,:)';
%X(t+1,:)=(A*X(t,:)'+B*U(t,:))';
end
k = K(:,:,N);

== matlab function PMSM_PI/Algorithm/电流环LQR/MATLAB Function2 ==
  data: P input; k output; Flux input; J input; Rs input; Ls input; B input; we input
function k  = fcn(P,Flux,J,Rs,Ls,B,we)

%A = [1-T*B/J 0 T*3*P*Flux/2/J;0 1-T-Rs/Ls T*we;-T*P*Flux/Ls -T*we 1-T*Rs/Ls];  %3*3
%B = [0 0;T/Ls 0;0 T/Ls];  %3*2
A = [-B/J 0 3*P*Flux/2/J;0 -Rs/Ls we;-P*Flux/Ls -we -Rs/Ls];  %3*3
B = [0 0;1/Ls 0;0 1/Ls];  %3*2
C = [1 0 0;0 1 0;0 0 1];  %3*3
D = 0;  %3*2  zeros(3,2)

Q = [100 0 0;0 10 0;0 0 10];  %3*3
R = [0.1 0;0 0.1];  %2*2

%X0=[];
N = 5;  %迭代次数
P = zeros(3,3,N+1);  %P的初始化,N+1个3*3的二维数组
P(:,:,N+1) = Q; %P的最后一个值为Q  P(:,:,2)=Q

for t=2:(N+1)  %t从2到21
    tused = (N+3-t);  %tused从21到2
    P(:,:,tused-1) = Q + A'*P(:,:,tused)*A-A'*P(:,:,tused)*B/(R+B'*P(:,:,tused)*B)*B'*P(:,:,tused)*A;  %黎卡提方程P的值为3*3   P(:,:,1)
end

K = zeros(2,3,N);  %初始化20*3

%U = zeros(N,2);  %初始化20*2
%X(1,:) = X0;

for t=1:N  %从1到20
K(:,:,t)=-(R+B'*P(:,:,t+1)*B)\B'*P(:,:,t+1)*A; %2*3
%U(t,:)=K(t,:)*X(t,:)';
%X(t+1,:)=(A*X(t,:)'+B*U(t,:))';
end
k = K(:,:,N);

== matlab function PMSM_PI/Algorithm/转速环电流环LQR消除静差/MATLAB Function1 ==
  data: k output; Rs input; Ls input; we input; I output; Flux input; J input; e output; xa input; u output
function [k,I,e,u] = fcn(Rs,Ls,we,Flux,J,xa)

T = 0.0001;
% A = [1-T*B/J 0 T*3*P*Flux/2/J;0 1-T*Rs/Ls T*we;-T*P*Flux/Ls -T*we 1-T*Rs/Ls];  %3*3
% B = [0 0;T/Ls 0;0 T/Ls];  %3*2

A = [1 0 T*3*5*Flux/2/J 0 0 -T*3*5*Flux/2/J;0 1-T*Rs/Ls T*we 0 T*Rs/Ls -T*we;-T*5*Flux/Ls -T*we 1-T*Rs/Ls T*5*Flux/Ls T*we T*Rs/Ls;0 0 0 1 0 0;0 0 0 0 1 0;0 0 0 0 0 1];  
B = [0 0;T/Ls 0;0 T/Ls;0 0;0 0;0 0];
Aa = [1 0 T*3*5*Flux/2/J;0 1-T*Rs/Ls T*we;-T*5*Flux/Ls -T*we 1-T*Rs/Ls];
Ba = [0 0;T/Ls 0;0 T/Ls];
xd = [xa(4) xa(5) xa(6)]';
% A = [1 0 3*5*Flux/2/J 0 0 0;0 1-T*Rs/Ls T*we 0 0 0;-T*5*Flux/Ls -T*we 1-T*Rs/Ls 0 0 0;0 0 0 1 0 0;0 0 0 0 1 0;0 0 0 0 0 1];  
% B = [0 0;T/Ls 0;0 T/Ls;0 0;0 0;0 0];

% A = [-Rs/Ls we 0 0;-we -Rs/Ls 0 0;0 0 1 0;0 0 0 1];  %2*2
% B = [1/Ls 0;0 1/Ls;0 0;0 0];  %2*2
% A = [-Rs/Ls we;-we -Rs/Ls];  %2*2
% B = [1/Ls 0;0 1/Ls];  %2*2
Qa = [1 0 0;0 10 0;0 0 100];
Ca = [1 0 0 -1 0 0;0 1 0 0 -1 0;0 0 1 0 0 -1];
Q = Ca'*Qa*Ca;  
R = [0.1 0;0 0.1];  %2*2

PN = Q;
err = 0.1;
error = 2;
i = 0;
while(error>err)
    PN_1 = Q + A'*PN*A-A'*PN*B/(R+B'*PN*B)*B'*PN*A;
    error = norm(PN-PN_1);
    PN = PN_1;
    i = i+1;
    if i>100
        break;
    end
end
P = PN;
K = -(R+B'*P*B)\B'*P*A;

ud = mldivide(Ba,(eye(3)-Aa)*xd);
u = K*xa+ud;
k = K;
I = i;
e = error;

== stateflow chart PMSM_PI/Algorithm/Chart1 ==
  state Out = Over_judge(Input) [function]
  state Out = Low_judge(Input) [function]
  state None
    during:
    Over_V= Over_judge(Udc);
    Low_V= Low_judge(Udc);
    STOP=Low_V+Over_V;
    exit:
    Over_V= Over_judge(Udc);
    Low_V= Low_judge(Udc);
    STOP=Low_V+Over_V;
  state Out
    during:
    Over_V=Over_judge(Udc);
    Low_V= Low_judge(Udc);
    STOP=Low_V+Over_V;
    Go = 1;
  (default) -> None : {up_limit = 28;down_limit = 15;}
  None -> Out : [Go_Flag == 1 && STOP ==0 ]
  Out -> None [order 2] : [Go_Flag == 0 ]
  Out -> None [order 1] : [ Over_V ==1|| Low_V==1]{Go = 0}
  data: Input function_input single size=1; Out function_output single; Input function_input single size=1; Out function_output single; Go_Flag input; Udc input; Over_V output single size=1 =0; STOP output single =0; Low_V output single size=1 =0; down_limit local; up_limit local; Time_count local single; Ts constant double =Ts; Go output =0

== matlab function PMSM_PI/Algorithm/电流环LQR/MATLAB Function1 ==
  data: k output; Rs input; Ls input; we input
function k   = fcn(Rs,Ls,we)

%A = [1-T*B/J 0 T*3*P*Flux/2/J;0 1-T-Rs/Ls T*we;-T*P*Flux/Ls -T*we 1-T*Rs/Ls];  %3*3
%B = [0 0;T/Ls 0;0 T/Ls];  %3*2
A = [-Rs/Ls we;-we -Rs/Ls];  %2*2
B = [1/Ls 0;0 1/Ls];  %3*2

Q = [10 0;0 10];  %3*3
R = [0.1 0;0 0.1];  %2*2

PN_1 = zeros(2,2);
PN = Q;
err = 0.01;
error = 1;
i = 0;
while(error>err)
    PN_1 = Q + A'*PN*A-A'*PN*B/(R+B'*PN*B)*B'*PN*A;
    error = norm(PN-PN_1);
    PN = PN_1;
    i = i+1;
    if i>100
        break;
    end
end
P = PN;
K = -(R+B'*P*B)\B'*P*A;

k = K;

== matlab function PMSM_PI/Algorithm/双环LQR/MATLAB Function1 ==
  data: P input; k output; Flux input; J input; Rs input; Ls input; B input; we input
function k   = fcn(P,Flux,J,Rs,Ls,B,we)

%A = [1-T*B/J 0 T*3*P*Flux/2/J;0 1-T-Rs/Ls T*we;-T*P*Flux/Ls -T*we 1-T*Rs/Ls];  %3*3
%B = [0 0;T/Ls 0;0 T/Ls];  %3*2
A = [-B/J 0 3*P*Flux/2/J;0 -Rs/Ls we;-P*Flux/Ls -we -Rs/Ls];  %3*3
B = [0 0;1/Ls 0;0 1/Ls];  %3*2
C = [1 0 0;0 1 0;0 0 1];  %3*3
D = 0;  %3*2  zeros(3,2)

Q = [1000 0 0;0 1 0;0 0 1];  %3*3
R = [0.1 0;0 0.1];  %2*2

PN_1 = zeros(3,3);
PN = Q;
err = 0.01;
error = 1;
i = 0;
while(error>err)
    PN_1 = Q + A'*PN*A-A'*PN*B/(R+B'*PN*B)*B'*PN*A;
    error = norm(PN-PN_1);
    PN = PN_1;
    i = i+1;
    if i>100
        break;
    end
end
P = PN;
K = -(R+B'*P*B)\B'*P*A;

k = K;
